simulink model "control_system"  (R2026b)
settings: Solver=ode4  StopTime=Tend  FixedStep=Ts
values from neighbouring files (symbols this model uses):
  pv = quad_params([],C(i).tauhat,C(i).ndhat)    [setup_simulink.m]    (also in validate_simulink_model.m = quad_params())
  pvt = quad_params();if scen==4,pvt=quad_params([1.3 1.3 2],1.5*pvt(16),pvt(17));end    [setup_simulink.m]
  Ts = S.Ts    [setup_simulink.m]
undefined symbols (not defined in the file or in its folder): G, kind, scen, sig
settings Model: Creator=XuanQuy  LastModifiedBy=XuanQuy
settings DataIOCC: SaveOutput=off  SaveTime=off  SignalLogging=off

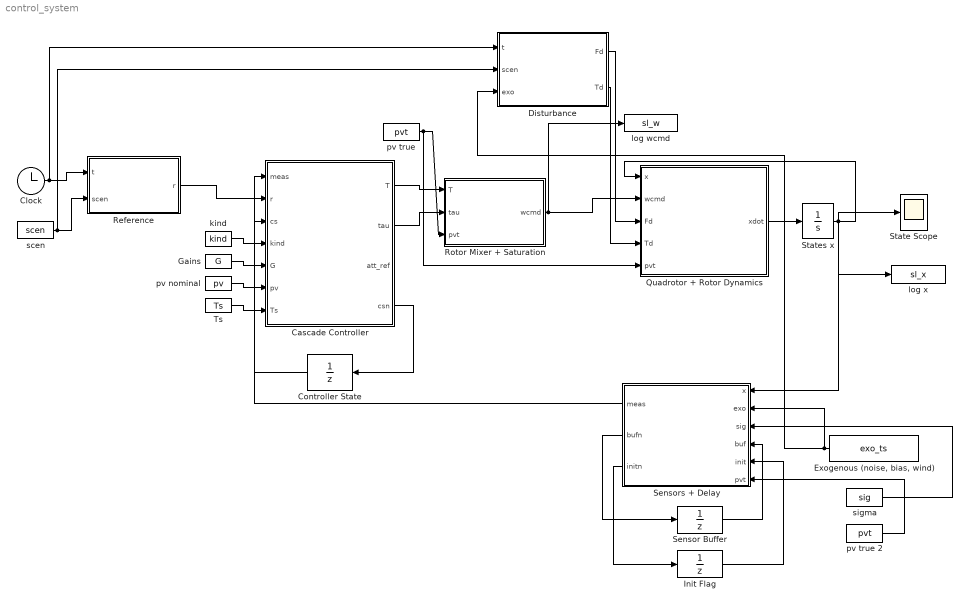
== system control_system ==
  Cascade Controller : MATLAB Function  TreatAsAtomicUnit=on  SystemSampleTime=Ts
  Clock : Clock
  Controller State : UnitDelay  InitialCondition=zeros(96,1)  SampleTime=Ts
  Disturbance : MATLAB Function  TreatAsAtomicUnit=on  SystemSampleTime=Ts
  "Exogenous (noise, bias, wind)" : FromWorkspace  VariableName=exo_ts  SampleTime=Ts  Interpolate=off  OutputAfterFinalValue=Holding final value
  Gains : Constant  Value=G
  Init Flag : UnitDelay  SampleTime=Ts
  Quadrotor + Rotor Dynamics : MATLAB Function  TreatAsAtomicUnit=on
  Reference : MATLAB Function  TreatAsAtomicUnit=on  SystemSampleTime=Ts
  Rotor Mixer + Saturation : MATLAB Function  TreatAsAtomicUnit=on  SystemSampleTime=Ts
  Sensor Buffer : UnitDelay  InitialCondition=zeros(12,11)  SampleTime=Ts
  Sensors + Delay : MATLAB Function  TreatAsAtomicUnit=on  SystemSampleTime=Ts
  State Scope : Scope
  States x : Integrator  InitialCondition=[zeros(12,1); sqrt(pvt(1)*pvt(2)/(4*pvt(4)))*ones(4,1)]
  Ts : Constant  Value=Ts
  kind : Constant  Value=kind
  log wcmd : ToWorkspace  VariableName=sl_w  SampleTime=Ts
  log x : ToWorkspace  VariableName=sl_x  SampleTime=Ts
  pv nominal : Constant  Value=pv
  pv true : Constant  Value=pvt
  pv true 2 : Constant  Value=pvt
  scen : Constant  Value=scen
  sigma : Constant  Value=sig
  wires:
  Clock/1 -> Reference/1(t), Disturbance/1(t)
  scen/1 -> Reference/2(scen), Disturbance/2(scen)
  "Exogenous (noise, bias, wind)"/1 -> Disturbance/3(exo), Sensors + Delay/2(exo)
  Sensors + Delay/1(meas) -> Cascade Controller/1(meas)
  Reference/1(r) -> Cascade Controller/2(r)
  Controller State/1 -> Cascade Controller/3(cs)
  kind/1 -> Cascade Controller/4(kind)
  Gains/1 -> Cascade Controller/5(G)
  pv nominal/1 -> Cascade Controller/6(pv)
  Ts/1 -> Cascade Controller/7(Ts)
  Cascade Controller/4(csn) -> Controller State/1
  Cascade Controller/1(T) -> Rotor Mixer + Saturation/1(T)
  Cascade Controller/2(tau) -> Rotor Mixer + Saturation/2(tau)
  pv true/1 -> Rotor Mixer + Saturation/3(pvt), Quadrotor + Rotor Dynamics/5(pvt)
  Rotor Mixer + Saturation/1(wcmd) -> Quadrotor + Rotor Dynamics/2(wcmd), log wcmd/1
  Disturbance/1(Fd) -> Quadrotor + Rotor Dynamics/3(Fd)
  Disturbance/2(Td) -> Quadrotor + Rotor Dynamics/4(Td)
  Quadrotor + Rotor Dynamics/1(xdot) -> States x/1
  States x/1 -> Quadrotor + Rotor Dynamics/1(x), State Scope/1, log x/1, Sensors + Delay/1(x)
  sigma/1 -> Sensors + Delay/3(sig)
  Sensor Buffer/1 -> Sensors + Delay/4(buf)
  Init Flag/1 -> Sensors + Delay/5(init)
  pv true 2/1 -> Sensors + Delay/6(pvt)
  Sensors + Delay/2(bufn) -> Sensor Buffer/1
  Sensors + Delay/3(initn) -> Init Flag/1

== matlab function control_system/Disturbance ==
  data: t input; Fd output; scen input; exo input; Td output
function [Fd, Td] = fcn(t, scen, exo)
%#codegen
[Fd, Td] = disturbance_gen(t, scen);
Fd = Fd + exo(16:18);

== matlab function control_system/Reference ==
  data: t input; r output; scen input
function r = fcn(t, scen)
%#codegen
r = reference_gen(t, scen);

== matlab function control_system/Cascade Controller ==
  data: meas input; T output; r input; cs input; kind input; G input; pv input; Ts input; tau output; att_ref output; csn output
function [T, tau, att_ref, csn] = fcn(meas, r, cs, kind, G, pv, Ts)
%#codegen
[T, tau, att_ref, csn] = ctrl_law(kind, G, cs, meas, r, pv, Ts);

== matlab function control_system/Rotor Mixer + Saturation ==
  data: T input; wcmd output; tau input; pvt input
function wcmd = fcn(T, tau, pvt)
%#codegen
[wcmd, ~, ~] = quad_mixer(T, tau, pvt);

== matlab function control_system/Quadrotor + Rotor Dynamics ==
  data: x input; xdot output; wcmd input; Fd input; Td input; pvt input
function xdot = fcn(x, wcmd, Fd, Td, pvt)
%#codegen
xdot = quad_dynamics(x, wcmd, Fd, Td, pvt);

== matlab function control_system/Sensors + Delay ==
  data: x input; meas output; exo input; sig input; buf input; init input; pvt input; bufn output; initn output
function [meas, bufn, initn] = fcn(x, exo, sig, buf, init, pvt)
%#codegen
[meas, bufn, initn] = sensor_buffer(x, exo(1:12), sig, exo(13:15), buf, init, pvt(17));
